simulink model "pmsm_plant"  (R2026b)
settings: Solver=VariableStepAuto  StopTime=6
values from neighbouring files (symbols this model uses):
  D = 5e-5    (= 5e-05)    [setup_motor.m]
  J = 0.0239    [setup_motor.m]
  L = (Ld + Lq) / 2    (= 0.000225)    [setup_motor.m]
  P = 10    [setup_motor.m]
  phi_m = 0.05867    [setup_motor.m]
  Rs = 25.68e-3    (= 0.02568)    [setup_motor.m]
  V_pico = 48    [setup_motor.m]
libraries: simulink x1
settings Model: Creator=Lemão Som  LastModifiedBy=Lemão Som

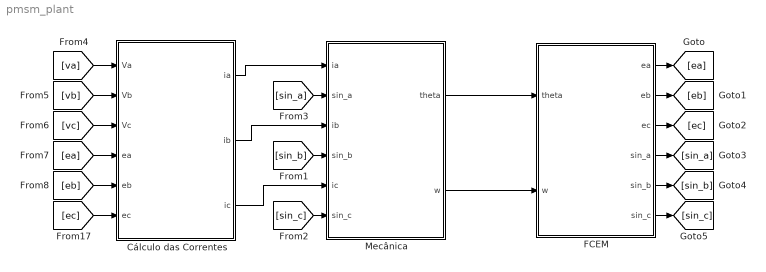
== system pmsm_plant ==
  Cálculo das Correntes : Subsystem
  FCEM : Subsystem
  Mecânica : Subsystem
  wires:
  Mecânica/2(w) -> FCEM/2(w)
  FCEM/2(eb) -> [eb]
  FCEM/5(sin_b) -> [sin_b]
  FCEM/1(ea) -> [ea]
  FCEM/4(sin_a) -> [sin_a]
  [vc] -> Cálculo das Correntes/3(Vc)
  [ea] -> Cálculo das Correntes/4(ea)
  [vb] -> Cálculo das Correntes/2(Vb)
  Mecânica/1(theta) -> FCEM/1(theta)
  [ec] -> Cálculo das Correntes/6(ec)
  [sin_b] -> Mecânica/4(sin_b)
  [va] -> Cálculo das Correntes/1(Va)
  [eb] -> Cálculo das Correntes/5(eb)
  Cálculo das Correntes/2(ib) -> Mecânica/3(ib)
  FCEM/6(sin_c) -> [sin_c]
  [sin_a] -> Mecânica/2(sin_a)
  FCEM/3(ec) -> [ec]
  Cálculo das Correntes/3(ic) -> Mecânica/5(ic)
  [sin_c] -> Mecânica/6(sin_c)
  Cálculo das Correntes/1(ia) -> Mecânica/1(ia)

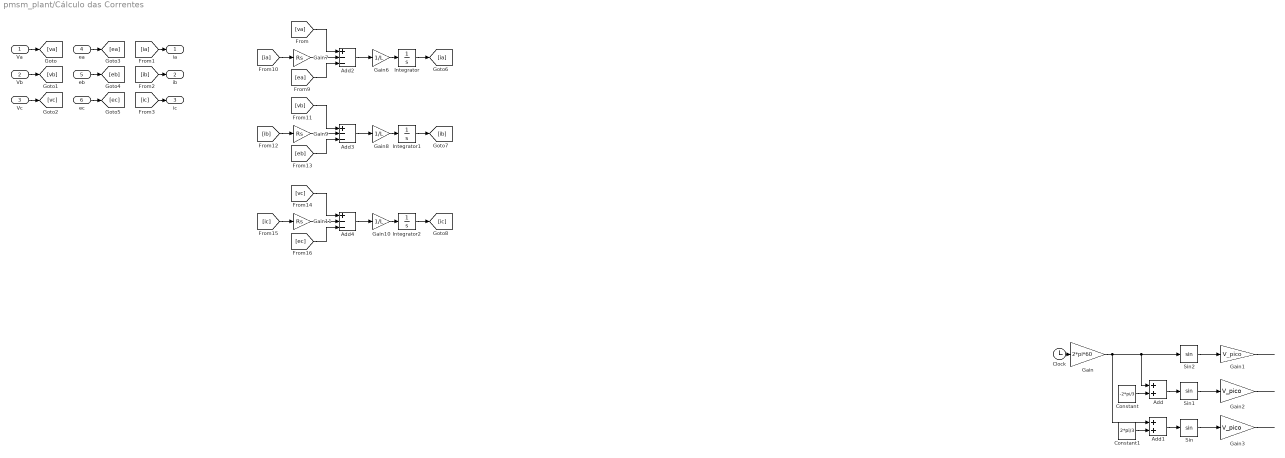
== system pmsm_plant/Cálculo das Correntes ==
  Va : Inport
  Vb : Inport  Port=2
  Vc : Inport  Port=3
  ea : Inport  Port=4
  eb : Inport  Port=5
  ec : Inport  Port=6
  Add : Sum
  Add1 : Sum
  Add2 : Sum  Inputs=+--
  Add3 : Sum  Inputs=+--
  Add4 : Sum  Inputs=+--
  Clock : Clock
  Constant : Constant  Value=-2*pi/3
  Constant1 : Constant  Value=2*pi/3
  Gain : Gain  Gain=2*pi*60
  Gain1 : Gain  Gain=V_pico
  Gain10 : Gain  Gain=1/L
  Gain11 : Gain  Gain=Rs
  Gain2 : Gain  Gain=V_pico
  Gain3 : Gain  Gain=V_pico
  Gain6 : Gain  Gain=1/L
  Gain7 : Gain  Gain=Rs
  Gain8 : Gain  Gain=1/L
  Gain9 : Gain  Gain=Rs
  Integrator : Integrator
  Integrator1 : Integrator
  Integrator2 : Integrator
  Sin : Trigonometry
  Sin1 : Trigonometry
  Sin2 : Trigonometry
  ia : Outport
  ib : Outport  Port=2
  ic : Outport  Port=3
  wires:
  Sin/1 -> Gain3/1
  Clock/1 -> Gain/1
  Gain1/1 -> ?
  Sin1/1 -> Gain2/1
  Gain2/1 -> ?
  Add1/1 -> Sin/1
  Sin2/1 -> Gain1/1
  Gain/1 -> Add/1, Sin2/1, Add1/1
  Gain3/1 -> ?
  Add/1 -> Sin1/1
  Constant/1 -> Add/2
  Constant1/1 -> Add1/2
  Integrator2/1 -> [ic]
  [ea] -> Add2/3
  [ec] -> Add4/3
  Add3/1 -> Gain8/1
  [eb] -> Add3/3
  Integrator1/1 -> [ib]
  Gain7/1 -> Add2/2
  Gain8/1 -> Integrator1/1
  Add4/1 -> Gain10/1
  Add2/1 -> Gain6/1
  Gain10/1 -> Integrator2/1
  [va] -> Add2/1
  [ic] -> Gain11/1
  Gain9/1 -> Add3/2
  [ia] -> Gain7/1
  Integrator/1 -> [ia]
  Gain11/1 -> Add4/2
  [vc] -> Add4/1
  [vb] -> Add3/1
  Gain6/1 -> Integrator/1
  [ib] -> Gain9/1
  Va/1 -> [va]
  Vb/1 -> [vb]
  Vc/1 -> [vc]
  ea/1 -> [ea]
  eb/1 -> [eb]
  ec/1 -> [ec]
  [ib] -> ib/1
  [ic] -> ic/1
  [ia] -> ia/1

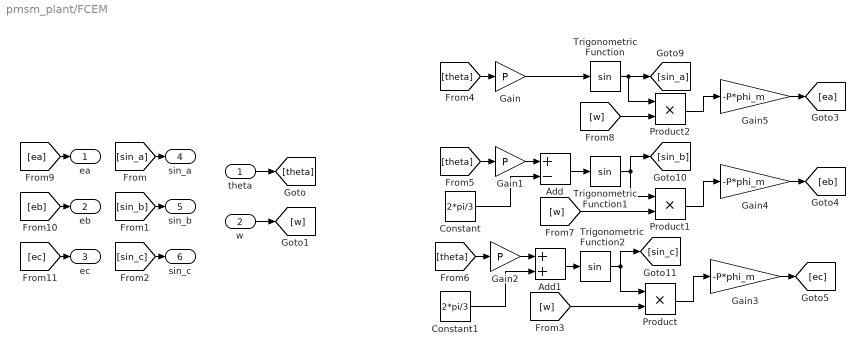
== system pmsm_plant/FCEM ==
  theta : Inport
  w : Inport  Port=2
  Add : Sum  Inputs=+-
  Add1 : Sum
  Constant : Constant  Value=2*pi/3
  Constant1 : Constant  Value=2*pi/3
  Gain : Gain  Gain=P
  Gain1 : Gain  Gain=P
  Gain2 : Gain  Gain=P
  Gain3 : Gain  Gain=-P*phi_m
  Gain4 : Gain  Gain=-P*phi_m
  Gain5 : Gain  Gain=-P*phi_m
  Product : Product
  Product1 : Product
  Product2 : Product
  Trigonometric Function : Trigonometry
  Trigonometric Function1 : Trigonometry
  Trigonometric Function2 : Trigonometry
  ea : Outport
  eb : Outport  Port=2
  ec : Outport  Port=3
  sin_a : Outport  Port=4
  sin_b : Outport  Port=5
  sin_c : Outport  Port=6
  wires:
  Product1/1 -> Gain4/1
  Gain5/1 -> [ea]
  Gain1/1 -> Add/1
  [theta] -> Gain/1
  Constant/1 -> Add/2
  Constant1/1 -> Add1/2
  Gain2/1 -> Add1/1
  Trigonometric Function/1 -> Product2/1, [sin_a]
  Trigonometric Function1/1 -> [sin_b], Product1/1
  Gain/1 -> Trigonometric Function/1
  Product/1 -> Gain3/1
  [w] -> Product2/2
  [w] -> Product1/2
  [theta] -> Gain1/1
  Add1/1 -> Trigonometric Function2/1
  Gain4/1 -> [eb]
  [theta] -> Gain2/1
  [w] -> Product/2
  Gain3/1 -> [ec]
  Product2/1 -> Gain5/1
  Add/1 -> Trigonometric Function1/1
  Trigonometric Function2/1 -> [sin_c], Product/1
  theta/1 -> [theta]
  w/1 -> [w]
  [ea] -> ea/1
  [eb] -> eb/1
  [ec] -> ec/1
  [sin_c] -> sin_c/1
  [sin_b] -> sin_b/1
  [sin_a] -> sin_a/1

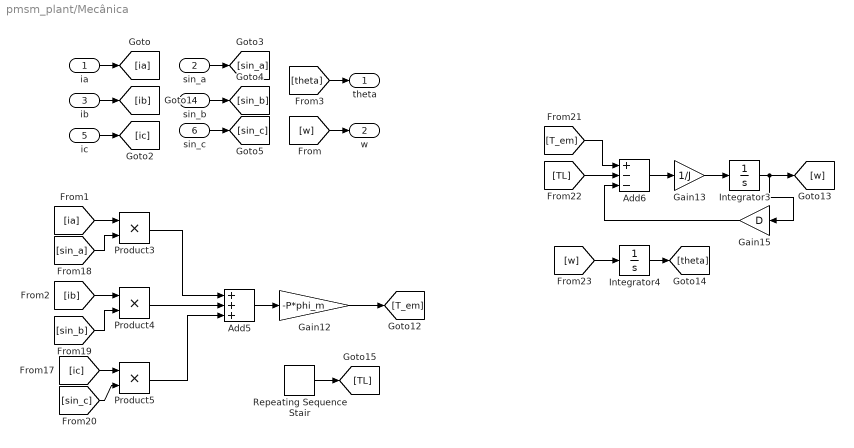
== system pmsm_plant/Mecânica ==
  ia : Inport
  sin_a : Inport  Port=2
  ib : Inport  Port=3
  sin_b : Inport  Port=4
  ic : Inport  Port=5
  sin_c : Inport  Port=6
  Add5 : Sum  Inputs=+++
  Add6 : Sum  Inputs=+--
  Gain12 : Gain  Gain=-P*phi_m
  Gain13 : Gain  Gain=1/J
  Gain15 : Gain  Gain=D
  Integrator3 : Integrator
  Integrator4 : Integrator
  Product3 : Product
  Product4 : Product
  Product5 : Product
  Repeating Sequence Stair : simulink/Sources/Repeating Sequence Stair  OutValues=[0, 0, 30, 60, 20, 0]  tsamp=1  OutMin=[]  OutMax=[]  OutDataTypeStr=double  OutputDataTypeScalingMode=double  OutDataType=fixdt(0,8)  ConRadixGroup=Best Precision: Vector-wise  OutScaling=2^-12
  theta : Outport
  w : Outport  Port=2
  wires:
  ic/1 -> [ic]
  ib/1 -> [ib]
  ia/1 -> [ia]
  [T_em] -> Add6/1
  [w] -> Integrator4/1
  [ia] -> Product3/1
  [ib] -> Product4/1
  [ic] -> Product5/1
  Product5/1 -> Add5/3
  [sin_b] -> Product4/2
  Integrator3/1 -> Gain15/1, [w]
  Gain15/1 -> Add6/3
  [sin_c] -> Product5/2
  [sin_a] -> Product3/2
  Add6/1 -> Gain13/1
  Add5/1 -> Gain12/1
  Integrator4/1 -> [theta]
  Gain13/1 -> Integrator3/1
  Repeating Sequence Stair/1 -> [TL]
  Product3/1 -> Add5/1
  [TL] -> Add6/2
  Gain12/1 -> [T_em]
  Product4/1 -> Add5/2
  sin_a/1 -> [sin_a]
  sin_b/1 -> [sin_b]
  sin_c/1 -> [sin_c]
  [theta] -> theta/1
  [w] -> w/1
